simulink model "case_12_slow_but_far"  (R2025b)
settings: Solver=VariableStepAuto  StartTime=0.0  StopTime=90  RelTol=1e-3
settings Model: Creator=sanborkl  LastModifiedBy=sanborkl

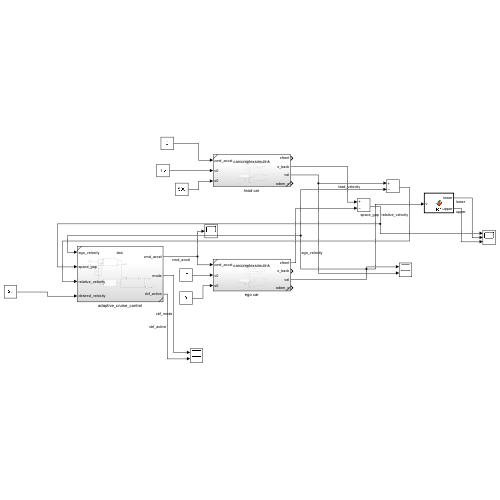
[thumbnail: Simulink's stored preview of the top-level diagram]
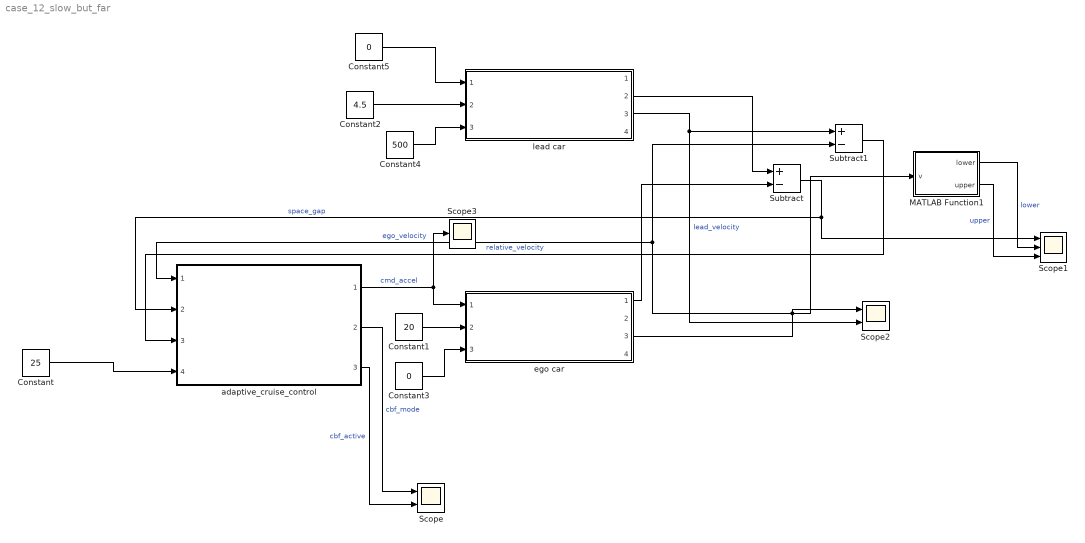
== system case_12_slow_but_far ==
  Constant : Constant  Value=25
  Constant1 : Constant  Value=20
  Constant2 : Constant  Value=4.5
  Constant3 : Constant  Value=0
  Constant4 : Constant  Value=500
  Constant5 : Constant  Value=0
  MATLAB Function1 : MATLAB Function  TreatAsAtomicUnit=on
  Scope : Scope  NumInputPorts=2
      settings: ActiveDisplayYMinimum=0.875  ActiveDisplayYMaximum=2.125
  Scope1 : Scope  NumInputPorts=3
      settings: ActiveDisplayYMinimum=-46.111520308404046  ActiveDisplayYMaximum=555.96794670093379  YLabel=m
  Scope2 : Scope  NumInputPorts=2
      settings: ActiveDisplayYMinimum=3.037745668052819  ActiveDisplayYMaximum=21.277314592684782  YLabel=m/s  DataLoggingVariableName=ScopeData2
  Scope3 : Scope
      settings: ActiveDisplayYMinimum=-1.76823896707685  ActiveDisplayYMaximum=1.8631376630085388  YLabel=m/s^2  DataLoggingVariableName=ScopeData3
  Subtract : Sum  Inputs=+-
  Subtract1 : Sum  Inputs=+-
  adaptive_cruise_control : Subsystem  ReferencedSubsystem=acc
  ego car : Subsystem  ReferencedSubsystem=carcomplexsimulink
  lead car : Subsystem  ReferencedSubsystem=carcomplexsimulink
  wires:
  ego car/3 -> Subtract1/2, adaptive_cruise_control/1, Scope2/1, MATLAB Function1/1(v)  "ego_velocity"
  adaptive_cruise_control/1 -> ego car/1, Scope3/1  "cmd_accel"
  Constant1/1 -> ego car/2
  Subtract1/1 -> adaptive_cruise_control/3  "relative_velocity"
  lead car/3 -> Scope2/2, Subtract1/1  "lead_velocity"
  Constant3/1 -> ego car/3
  Constant2/1 -> lead car/2
  adaptive_cruise_control/2 -> Scope/1  "cbf_mode"
  lead car/2 -> Subtract/1
  adaptive_cruise_control/3 -> Scope/2  "cbf_active"
  Constant/1 -> adaptive_cruise_control/4
  ego car/1 -> Subtract/2
  Subtract/1 -> Scope1/1, adaptive_cruise_control/2  "space_gap"
  Constant4/1 -> lead car/3
  Constant5/1 -> lead car/1
  MATLAB Function1/1(lower) -> Scope1/2  "lower"
  MATLAB Function1/2(upper) -> Scope1/3  "upper"

== matlab function case_12_slow_but_far/MATLAB Function1 ==
  data: v input; lower output; upper output
function [lower, upper] = fcn(v)

lower = 2 * v + 5;
upper = 2 * v + 15;
